simulink model "GasChargedAccumulatorTestRig"  (R2026b)
settings: Solver=VariableStepAuto  StopTime=12  MaxStep=0.24  AbsTol=1e-3  EnableMultiTasking=on
libraries: SimscapeFluids_lib x3, fl_lib x3, nesl_utility x3, simulink x2
CloseFcn:
  | try,close(h1_GasChargedAccumulatorTestRig),end
  | clear h1_GasChargedAccumulatorTestRig
  | 
  | clear simlog_GasChargedAccumulatorTestRig tout
settings Model: Creator=The MathWorks, Inc.  LastModifiedBy=grouleau
settings SolverCC: AutoScaleAbsTol=off
settings DataIOCC: LimitDataPoints=on  MaxDataPoints=10000  ReturnWorkspaceOutputs=off  SaveFormat=Array  SignalLoggingName=logsout_GasChargedAccumulatorTestRig
settings OptimizationCC: LifeSpan=inf  MemsetInitFltsAndDblsToZero=off
settings DebuggingCC: AllowSymbolicDim=off  ArithmeticOperatorsInVariantConditions=warning  MultiTaskCondExecSysMsg=none  MultiTaskDSMMsg=warning  PregeneratedLibrarySubsystemCodeDiagnostic=none  SFExecutionAtInitializationDiag=none  SFNoUnconditionalDefaultTransitionDiag=warning  SFUnexpectedBacktrackingDiag=warning  SaveWithParameterizedLinksMsg=none  SignalResolutionControl=TryResolveAllWithWarning  SolverPrmCheckMsg=warning  StateNameClashWarn=warning
settings HardwareCC: ProdEndianess=Unspecified  ProdHWDeviceType=32-bit Generic  ProdIntDivRoundTo=Undefined  ProdLargestAtomicFloat=None
settings ModelReferenceCC: PropagateSignalLabelsOutOfModel=off
settings SFSimCC: CustomCodeUndefinedFunction=UseInterfaceOnly  SimUseLocalCustomCode=off
settings RTWCC: DLArmComputeVersion=19.05  RTWUseLocalCustomCode=off
settings CodeAppCC: StateflowObjectComments=on
settings GRTTargetCC: CombineOutputUpdateFcns=off  GRTInterface=on  TargetFcnLib=ansi_tfl_tmw.mat  TargetLangStandard=C89/C90 (ANSI)
settings ConfigComp: CovExternalEMLEnable=off  CovSFcnEnable=off  CovSaveCumulativeToWorkspaceVar=on  CovSaveSingleToWorkspaceVar=on
settings SimscapeCC: SimscapeLogName=simlog_GasChargedAccumulatorTestRig  SimscapeLogSimulationStatistics=on  SimscapeLogType=all  SimscapeUseEnergyAccounting=off

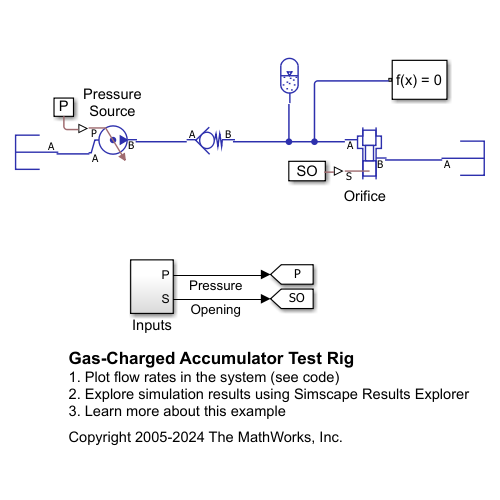
[thumbnail: Simulink's stored preview of the top-level diagram]
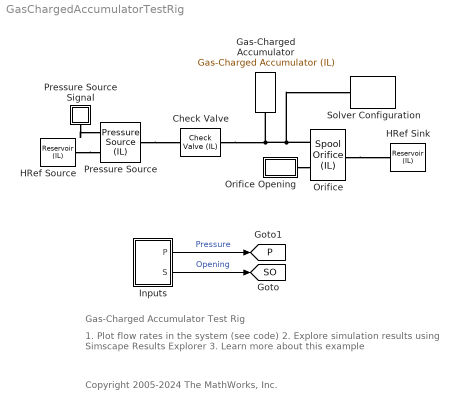
== system GasChargedAccumulatorTestRig ==
  note: Gas-Charged Accumulator Test Rig
  note: 1. Plot flow rates in the system (see code)
      | 2. Explore simulation results using Simscape Results Explorer
      | 3. Learn more about this example
  note: Copyright 2005-2024 The MathWorks, Inc.
  Check Valve : SimscapeFluids_lib/Isothermal Liquid/Valves & Orifices/Directional Control Valves/Check Valve (IL)  Tag=Factory Generic  opening_spec=fluids.isothermal_liquid.valves_orifices.enum.PressureOpeningSpec.Linear  pressure_control_spec=fluids.isothermal_liquid.valves_orifices.enum.pressure_control_spec.dp  p_crack_differential=0.03 MPa  p_crack_gauge=0.1 MPa  press_max_differential=0.12 MPa  press_max_gauge=0.2 MPa  area_max=0.0001 m^2  area_leak=1e-12 m^2  p_diff_TLU=[0.01 : 0.01 : 0.1] MPa  valve_area_TLU=[1e-10, 1e-05, 2e-05, 3e-05, 4e-05, 5e-05, 6e-05, 7.5e-05, 8.5e-05, .0001] m^2  vol_flow_TLU=[.000358, .045, .11, .191, .284, .39, .505, .63, .764, .905] .* 1e-3 m^3/s  area=inf m^2  Cd=0.7  Re_c=150  smoothing_factor=0  pressure_recovery=false  opening_dynamics=0  tau=0.1 s
      settings: LibrarySourceBlock=SimscapeFluids_lib/Isothermal Liquid/Valves & Orifices/Directional Control Valves/Check Valve (IL)
  Gas-Charged Accumulator : SimscapeFluids_lib/Isothermal Liquid/Tanks & Accumulators/Gas-Charged Accumulator (IL)  capacity=8 l  dead_volume=0.08 l  p_precharge=0.6 MPa  k_sh=1.4  stiff_coeff=1e12 Pa/m^3  dynamic_compressibility=simscape.enum.onoff.off  liquid_volume_specify=on  liquid_volume_priority=High  liquid_volume=1 l  liquid_volume_nominal_specify=off  liquid_volume_nominal_value=1  liquid_volume_nominal_unit=m^3  liquid_mass_specify=off  liquid_mass_priority=None  liquid_mass=5 kg  liquid_mass_nominal_specify=off  liquid_mass_nominal_value=1  liquid_mass_nominal_unit=kg  p_I_specify=on  p_I_priority=High  p_I=0.2 MPa  p_I_nominal_specify=off  p_I_nominal_value=1  p_I_nominal_unit=Pa
      settings: LibrarySourceBlock=SimscapeFluids_lib/Isothermal Liquid/Tanks & Accumulators/Gas-Charged Accumulator (IL)
  HRef Sink : fl_lib/Isothermal Liquid/Elements/Reservoir (IL)  Tag=Factory Generic  pressure_input=false  pressure_spec=foundation.enum.pressure_spec.atmospheric  reservoir_pressure=0.101325 MPa
  HRef Source : fl_lib/Isothermal Liquid/Elements/Reservoir (IL)  Tag=Factory Generic  pressure_input=false  pressure_spec=foundation.enum.pressure_spec.atmospheric  reservoir_pressure=0.101325 MPa
  Inputs : Subsystem
  Orifice : SimscapeFluids_lib/Isothermal Liquid/Valves & Orifices/Orifices/Spool Orifice (IL)  Tag=Factory Generic  orifice_spec=2  diameter_hole=5e-3 m  num_hole=6  width=0.02 m  del_S_max=1 m  S_min=0 m  open_orientation=1  flow_force_spec=false  clearance=1e-5 m  area_leak=1e-12 m^2  area=inf m^2  Cd=0.7  Re_c=150  smoothing_factor=0  pressure_recovery=false
  Orifice Opening : Subsystem
      mask Display: disp('SO');
  Pressure Source : fl_lib/Isothermal Liquid/Sources/Pressure Source (IL)  Tag=Factory Generic  source_type=foundation.enum.constant_controlled.controlled  pressure_differential=0 MPa
  Pressure Source Signal : Subsystem
      mask Display: disp('P')
  Solver Configuration : nesl_utility/Solver Configuration  PhysicalDomain=network_engine_domain  SubClassName=solver  LeftPortType=input  RightPortType=generic  Tones=[]  Harmonics=[]  SimulateNoise=off  Profile=off  UseLocalSampling=off  EnableSwitchedLinearOptims=on  FrequencyDomain=off  UseCCode=off  RelTol=0.001  AbsTol=1e-06  MinStep=1e-09  ToWorkspace=off  RevertToSquareIcSolve=off  NumHomotopyIterations=100  PhasorMode=off  PhasorModeNumHarmonics=1  ConsistencySolver=NEWTON_XTOL_AFTER_FTOL  CanonicalOrdering=UNORDERED  OptimizeIntermediates=UNOPTIMIZED  MulticoreSolverChoice=BACKWARD_EULER  IndexReductionMethod=DerivativeReplacement  DoDC=off  ResidualTolerance=1e-9  ConsistencyTolSource=GLOBAL  ConsistencyAbsTol=0.001  ConsistencyRelTol=0.001  ConsistencyTolFactor=0.001  UseLocalSolver=off  LocalSolverChoice=NE_BACKWARD_EULER_ADVANCER  ResolveIndetEquations=on  FunctionEvalNumThread=1  LocalSolverSampleTime=.001  DoFixedCost=off  MaxNonlinIter=3  MaxModeIter=2  ComputeImpulses=off  ImpulseIterations=2  LinearAlgebra=auto  LinearAlgebraNumThread=0  EquationFormulation=NE_TIME_EF  DelaysMemoryBudget=1024  AutomaticFiltering=on  FilteringTimeConstant=0.001  PartitionStorageMethod=AS_NEEDED  PartitionMemoryBudget=1024  PartitionMethod=FAST  MultibodyUseLocalSolver=off  MultibodyLocalSolverChoice=ODE1  MultibodyLocalSolverSampleTime=0.001
  tag scope: P=global, SO=global
  wires:
  Inputs/2(S) -> [SO]  "Opening"
  Inputs/1(P) -> [P]  "Pressure"
  connections:
  Orifice/LConn2 -- Solver Configuration/RConn1 -- Gas-Charged Accumulator/RConn1 -- Check Valve/RConn1
  Orifice/RConn1 -- HRef Sink/LConn1
  Orifice Opening/RConn1 -- Orifice/LConn1
  HRef Source/LConn1 -- Pressure Source/LConn1
  Pressure Source Signal/RConn1 -- Pressure Source/LConn2
  Pressure Source/RConn1 -- Check Valve/LConn1

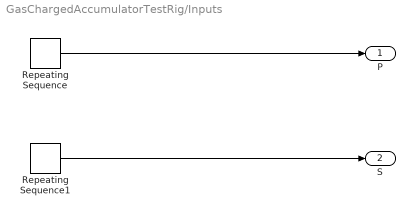
== system GasChargedAccumulatorTestRig/Inputs ==
  Repeating Sequence : simulink/Sources/Repeating Sequence  rep_seq_t=[0 0.2 2.8 3 6 6.2 8.8 9 12]  rep_seq_y=[500000 1000000 1000000 500000 500000 1000000 1000000 500000 500000]
  Repeating Sequence1 : simulink/Sources/Repeating Sequence  rep_seq_t=[0 3.5 3.7 5.3 5.5 9.5 9.7 11.3 11.5 12]  rep_seq_y=[0 0 0.005 0.00498 2e-05 0 0.00495 0.00495 0 0]
  P : Outport
  S : Outport  Port=2
  wires:
  Repeating Sequence/1 -> P/1
  Repeating Sequence1/1 -> S/1

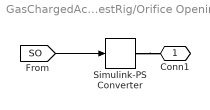
== system GasChargedAccumulatorTestRig/Orifice Opening ==
  Simulink-PS Converter : nesl_utility/Simulink-PS Converter  PhysicalDomain=network_engine_domain  SubClassName=ps_input  LeftPortType=input  RightPortType=output  PseudoPeriodic=off  Frequencies=[]  NoiseDistribution=none  NoiseParameters=[]  Unit=1  AffineConversion=off  FilteringAndDerivatives=zero  SimscapeFilterOrder=1  InputFilterTimeConstant=.001  UdotUserProvided=0
  Conn1 : PMIOPort  Side=Right
  wires:
  [SO] -> Simulink-PS Converter/1
  connections:
  Simulink-PS Converter/RConn1 -- Conn1/RConn1

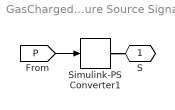
== system GasChargedAccumulatorTestRig/Pressure Source Signal ==
  Simulink-PS Converter1 : nesl_utility/Simulink-PS Converter  PhysicalDomain=network_engine_domain  SubClassName=ps_input  LeftPortType=input  RightPortType=output  PseudoPeriodic=off  Frequencies=[]  NoiseDistribution=none  NoiseParameters=[]  Unit=1  AffineConversion=off  FilteringAndDerivatives=zero  SimscapeFilterOrder=1  InputFilterTimeConstant=.001  UdotUserProvided=0
  S : PMIOPort  Side=Right
  wires:
  [P] -> Simulink-PS Converter1/1
  connections:
  Simulink-PS Converter1/RConn1 -- S/RConn1
